simulink subsystem "Subsys_GFormConv_InnerCtrl_cascadedPI"  (R2024b)
settings: Solver=VariableStepAuto  StartTime=0.0  StopTime=10.0  RelTol=1e-3
model mask{f_n=50, L_filter_conv_pu=[ 0.0001 0.05097], C_filter_pu=[ 0.06875 0.04569 ], send_info_messages=0, K_p_V_cap_controller=0.8, K_i_V_cap_controller=0.5, K_p_I_conv_controller=3.3, K_i_I_conv_controller=16.5, Cff_V_cap_ctrl=0, Cff_I_conv_ctrl=0, K_ff_I_grid=1, K_ff_V_cap=1, i_conv_limit=1, v_conv_limit=1.3, i_lim_type=0, T_s_ctrl=1e-4, T_s_PWM_meas=1e-4, datatype='double'}
  mask prompts: f_n "Nominal frequency [Hz]"; L_filter_conv_pu "Impedance of Converter-Side Inductor [ R L ] (p.u.)"; C_filter_pu "Impedance of Filter Capacitor [ R C ] (p.u.)"; send_info_messages "Send info messages when limiting reference values (0 = disabled, 1 = enabled)"; K_p_V_cap_controller "Voltage controller proportional gain [p.u.]"; K_i_V_cap_controller "Voltage controller integral gain [p.u.]"; K_p_I_conv_controller "Current controller proportional gain [p.u.]"; K_i_I_conv_controller "Current controller integral gain [p.u.]"; Cff_V_cap_ctrl "Command-feed-forward (voltage controller) (0 = disabled, 1 = enabled)"; Cff_I_conv_ctrl "Command-feed-forward (current controller) (0 = disabled, 1 = enabled)"; K_ff_I_grid "Current-feed-forward (voltage controller) (0 = disabled, 1 = enabled)"; K_ff_V_cap "Voltage-feed-forward (current controller) (0 = disabled, 1 = enabled)"; i_conv_limit "Converter current maximum value (limit) [p.u.]"; v_conv_limit "Converter voltage maximum value (limit) [p.u.]"; i_lim_type "Coordinate system of current setpoint limiter (0 = dq, 1 = abc)"; T_s_ctrl "Controller sample time [s]"; T_s_PWM_meas "PWM and measurements sample time [s]"; datatype "Signal data type"
libraries: simulink x8
settings Model: Creator=winkens  LastModifiedBy=k.kocaogullar
settings SolverCC: AlgebraicLoopSolver=TrustRegion
settings OptimizationCC: ReuseModelBlockBuffer=off
settings DebuggingCC: UnconnectedInputMsg=warning  UnconnectedOutputMsg=warning  UnconnectedLineMsg=warning
settings ModelReferenceCC: EnableRefExpFcnMdlSchedulingChecks=on
settings RTWCC: GPUComputeCapability=3.5  DLArmComputeVersion=19.05

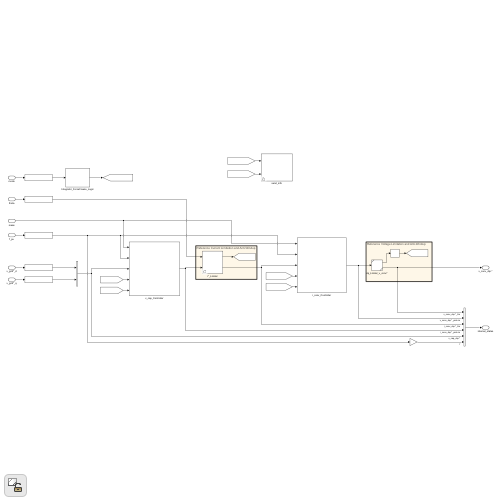
[thumbnail: Simulink's stored preview of the top-level diagram]
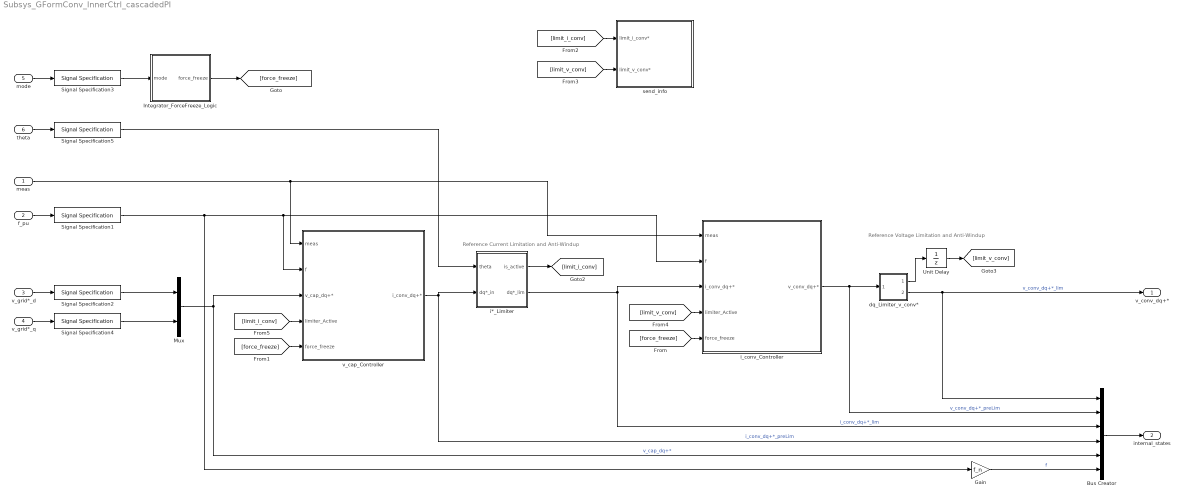
== system Subsys_GFormConv_InnerCtrl_cascadedPI ==
  note: Reference Current Limitation and Anti-Windup
  note: Reference Voltage Limitation and Anti-Windup
  meas : Inport
  f_pu : Inport  Port=2
  v_grid*_d : Inport  Port=3
  v_grid*_q : Inport  Port=4
  mode : Inport  Port=5
  theta : Inport  Port=6
  Bus Creator : BusCreator  Inputs=6
  Gain : Gain  Gain=f_n
  Integrator_ForceFreeze_Logic : Subsystem
  Mux : Mux  Inputs=2
  Signal Specification{1..4} (4 alike) : SignalSpecification  SampleTime=T_s_ctrl
  Signal Specification5 : SignalSpecification  SampleTime=T_s_PWM_meas
  Unit Delay : UnitDelay  SampleTime=-1  HasFrameUpgradeWarning=on
  dq_Limiter_v_conv* : Subsystem  ReferencedSubsystem=dq_Limiter  X_dq_max=v_conv_limit  datatype=datatype
  i*_Limiter : Subsystem  Variant=on  VariantControl=Choice
  "i_conv_Controller " : Subsystem
  send_info : Subsystem  Variant=on
  v_cap_Controller : Subsystem
  v_conv_dq+* : Outport
  internal_states : Outport  Port=2
  wires:
  Unit Delay/1 -> [limit_v_conv]
  Mux/1 -> Bus Creator/5, v_cap_Controller/3(v_cap_dq+*)  "v_cap_dq+*"
  v_grid*_d/1 -> Signal Specification2/1
  dq_Limiter_v_conv*/2 -> v_conv_dq+*/1, Bus Creator/1  "v_conv_dq+*_lim"
  f_pu/1 -> Signal Specification1/1
  v_cap_Controller/1(i_conv_dq+*) -> i*_Limiter/2(dq*_in), Bus Creator/4  "i_conv_dq+*_preLim"
  [force_freeze] -> "i_conv_Controller "/5(force_freeze)
  Gain/1 -> Bus Creator/6  "f"
  Signal Specification4/1 -> Mux/2
  dq_Limiter_v_conv*/1 -> Unit Delay/1
  "i_conv_Controller "/1(v_conv_dq+*) -> dq_Limiter_v_conv*/1, Bus Creator/2  "v_conv_dq+*_preLim"
  mode/1 -> Signal Specification3/1
  Bus Creator/1 -> internal_states/1
  meas/1 -> v_cap_Controller/1(meas), "i_conv_Controller "/1(meas)
  Signal Specification1/1 -> v_cap_Controller/2(f), "i_conv_Controller "/2(f), Gain/1
  Signal Specification2/1 -> Mux/1
  v_grid*_q/1 -> Signal Specification4/1
  theta/1 -> Signal Specification5/1
  i*_Limiter/1(is_active) -> [limit_i_conv]
  i*_Limiter/2(dq*_lim) -> Bus Creator/3, "i_conv_Controller "/3(i_conv_dq+*)  "i_conv_dq+*_lim"
  Signal Specification5/1 -> i*_Limiter/1(theta)
  [limit_i_conv] -> send_info/1(limit_i_conv*)
  [limit_v_conv] -> send_info/2(limit_v_conv*)
  Signal Specification3/1 -> Integrator_ForceFreeze_Logic/1(mode)
  Integrator_ForceFreeze_Logic/1(force_freeze) -> [force_freeze]
  [force_freeze] -> v_cap_Controller/5(force_freeze)
  [limit_v_conv] -> "i_conv_Controller "/4(limiter_Active)
  [limit_i_conv] -> v_cap_Controller/4(limiter_Active)

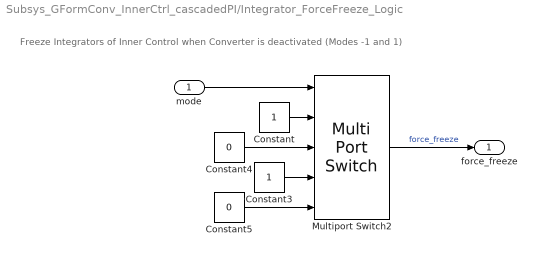
== system Subsys_GFormConv_InnerCtrl_cascadedPI/Integrator_ForceFreeze_Logic ==
  note: Freeze Integrators of Inner Control when Converter is deactivated (Modes -1 and 1)
  mode : Inport
  Constant : Constant  OutDataTypeStr=boolean
  Constant3 : Constant  OutDataTypeStr=boolean
  Constant4 : Constant  Value=0  OutDataTypeStr=boolean
  Constant5 : Constant  Value=0  OutDataTypeStr=boolean
  Multiport Switch2 : MultiPortSwitch  DataPortOrder=Specify indices  DataPortIndices={-1,0,1,2}  SaturateOnIntegerOverflow=off  InputSameDT=off
  force_freeze : Outport
  wires:
  Constant5/1 -> Multiport Switch2/5
  Constant4/1 -> Multiport Switch2/3
  Constant3/1 -> Multiport Switch2/4
  Constant/1 -> Multiport Switch2/2
  mode/1 -> Multiport Switch2/1
  Multiport Switch2/1 -> force_freeze/1  "force_freeze"

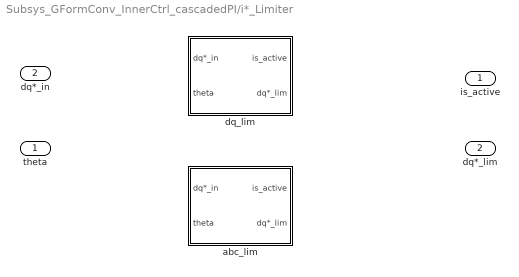
== system Subsys_GFormConv_InnerCtrl_cascadedPI/i*_Limiter ==
  theta : Inport
  dq*_in : Inport  Port=2
  abc_lim : Subsystem  VariantControl=i_lim_type > 0.5
  dq_lim : Subsystem  VariantControl=(default)
  is_active : Outport
  dq*_lim : Outport  Port=2

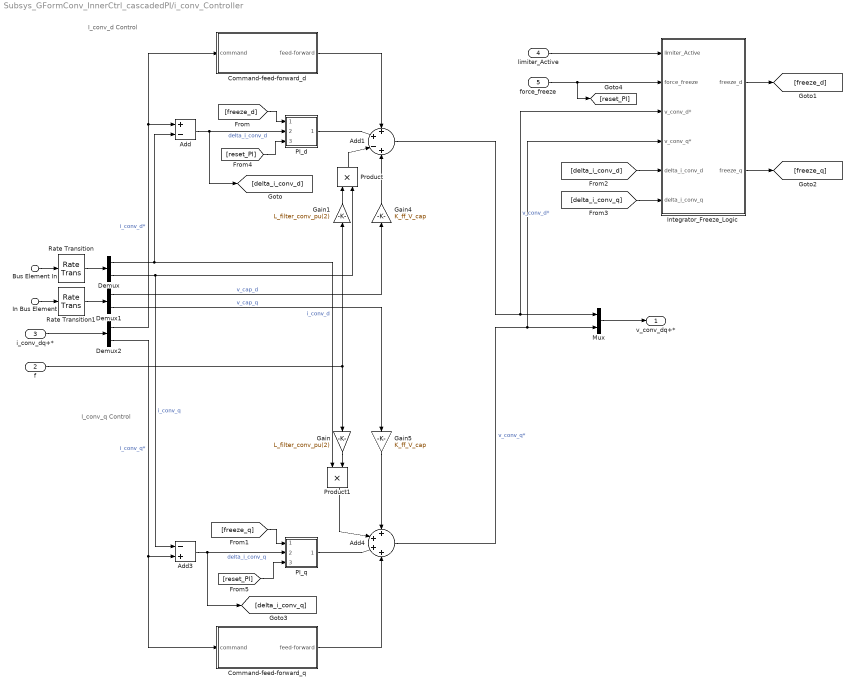
== system Subsys_GFormConv_InnerCtrl_cascadedPI/i_conv_Controller  ==
  note: I_conv_q Control
  note: I_conv_d Control
  Bus Element In : Inport  PortName=meas  Element=dq+.i_conv_dq+
  In Bus Element : Inport  PortName=meas  Element=dq+.v_cap_dq+
  f : Inport  Port=2
  i_conv_dq+* : Inport  Port=3
  limiter_Active : Inport  Port=4
  force_freeze : Inport  Port=5
  Add : Sum  Inputs=+-
  Add1 : Sum  Inputs=++-+
  Add3 : Sum  Inputs=-+
  Add4 : Sum  Inputs=++++
  Command-feed-forward_d : Subsystem  Variant=on  VariantControl=Choice
  Command-feed-forward_q : Subsystem  Variant=on  VariantControl=Choice
  Demux : Demux  Outputs=2
  Demux1 : Demux  Outputs=2
  Demux2 : Demux  Outputs=2
  Gain : Gain  Gain=L_filter_conv_pu(2)
  Gain1 : Gain  Gain=L_filter_conv_pu(2)
  Gain4 : Gain  Gain=K_ff_V_cap
  Gain5 : Gain  Gain=K_ff_V_cap
  Integrator_Freeze_Logic : Subsystem
  Mux : Mux  Inputs=2
  PI_d : Subsystem  ReferencedSubsystem=PI_freeze  K_p=K_p_I_conv_controller  K_i=K_i_I_conv_controller  T_s=T_s_ctrl  datatype=datatype
  PI_q : Subsystem  ReferencedSubsystem=PI_freeze  K_p=K_p_I_conv_controller  K_i=K_i_I_conv_controller  T_s=T_s_ctrl  datatype=datatype
  Product : Product  Inputs=**
  Product1 : Product  Inputs=**
  Rate Transition : RateTransition  Deterministic=off  OutPortSampleTime=T_s_ctrl
  Rate Transition1 : RateTransition  Deterministic=off  OutPortSampleTime=T_s_ctrl
  v_conv_dq+* : Outport
  wires:
  Add4/1 -> Integrator_Freeze_Logic/4(v_conv_q*), Mux/2  "v_conv_q*"
  Add3/1 -> PI_q/2, [delta_i_conv_q]  "delta_i_conv_q"
  Add1/1 -> Integrator_Freeze_Logic/3(v_conv_d*), Mux/1  "v_conv_d*"
  Product/1 -> Add1/3
  PI_q/1 -> Add4/3
  Mux/1 -> v_conv_dq+*/1
  Product1/1 -> Add4/2
  Gain1/1 -> Product/1
  Demux2/1 -> Add/1, Command-feed-forward_d/1(command)  "i_conv_d*"
  PI_d/1 -> Add1/2
  Demux/2 -> Add3/1, Product/2  "i_conv_q"
  f/1 -> Gain/1, Gain1/1
  Demux2/2 -> Command-feed-forward_q/1(command), Add3/2  "i_conv_q*"
  Demux1/2 -> Gain5/1  "v_cap_q"
  Bus Element In/1 -> Rate Transition/1
  i_conv_dq+*/1 -> Demux2/1
  Demux1/1 -> Gain4/1  "v_cap_d"
  Demux/1 -> Product1/1, Add/2  "i_conv_d"
  Add/1 -> PI_d/2, [delta_i_conv_d]  "delta_i_conv_d"
  In Bus Element/1 -> Rate Transition1/1
  Command-feed-forward_q/1(feed-forward) -> Add4/4
  Gain/1 -> Product1/2
  [freeze_d] -> PI_d/1
  [freeze_q] -> PI_q/1
  Gain4/1 -> Add1/4
  Gain5/1 -> Add4/1
  Command-feed-forward_d/1(feed-forward) -> Add1/1
  Rate Transition/1 -> Demux/1
  Rate Transition1/1 -> Demux1/1
  force_freeze/1 -> [reset_PI], Integrator_Freeze_Logic/2(force_freeze)
  Integrator_Freeze_Logic/1(freeze_d) -> [freeze_d]
  Integrator_Freeze_Logic/2(freeze_q) -> [freeze_q]
  limiter_Active/1 -> Integrator_Freeze_Logic/1(limiter_Active)
  [delta_i_conv_d] -> Integrator_Freeze_Logic/5(delta_i_conv_d)
  [delta_i_conv_q] -> Integrator_Freeze_Logic/6(delta_i_conv_q)
  [reset_PI] -> PI_d/3
  [reset_PI] -> PI_q/3

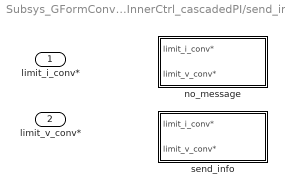
== system Subsys_GFormConv_InnerCtrl_cascadedPI/send_info ==
  limit_i_conv* : Inport
  limit_v_conv* : Inport  Port=2
  no_message : Subsystem  VariantControl=(default)
  send_info : Subsystem  VariantControl=send_info_messages > 0.5

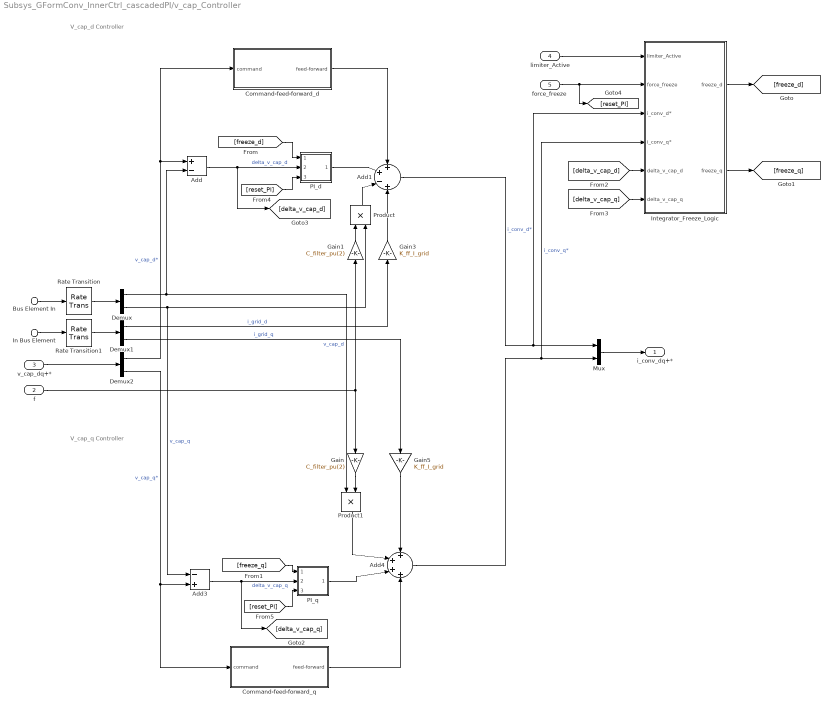
== system Subsys_GFormConv_InnerCtrl_cascadedPI/v_cap_Controller ==
  note: V_cap_q Controller
  note: V_cap_d Controller
  Bus Element In : Inport  PortName=meas  Element=dq+.v_cap_dq+
  In Bus Element : Inport  PortName=meas  Element=dq+.i_filter_grid_dq+
  f : Inport  Port=2
  v_cap_dq+* : Inport  Port=3
  limiter_Active : Inport  Port=4
  force_freeze : Inport  Port=5
  Add : Sum  Inputs=+-
  Add1 : Sum  Inputs=++-+
  Add3 : Sum  Inputs=-+
  Add4 : Sum  Inputs=++++
  Command-feed-forward_d : Subsystem  Variant=on  VariantControl=Choice
  Command-feed-forward_q : Subsystem  Variant=on  VariantControl=Choice
  Demux : Demux  Outputs=2
  Demux1 : Demux  Outputs=2
  Demux2 : Demux  Outputs=2
  Gain : Gain  Gain=C_filter_pu(2)
  Gain1 : Gain  Gain=C_filter_pu(2)
  Gain3 : Gain  Gain=K_ff_I_grid
  Gain5 : Gain  Gain=K_ff_I_grid
  Integrator_Freeze_Logic : Subsystem
  Mux : Mux  Inputs=2
  PI_d : Subsystem  ReferencedSubsystem=PI_freeze  K_p=K_p_V_cap_controller  K_i=K_i_V_cap_controller  T_s=T_s_ctrl  datatype=datatype
  PI_q : Subsystem  ReferencedSubsystem=PI_freeze  K_p=K_p_V_cap_controller  K_i=K_i_V_cap_controller  T_s=T_s_ctrl  datatype=datatype
  Product : Product  Inputs=**
  Product1 : Product  Inputs=**
  Rate Transition : RateTransition  Deterministic=off  OutPortSampleTime=T_s_ctrl
  Rate Transition1 : RateTransition  Deterministic=off  OutPortSampleTime=T_s_ctrl
  i_conv_dq+* : Outport
  wires:
  Bus Element In/1 -> Rate Transition/1
  In Bus Element/1 -> Rate Transition1/1
  v_cap_dq+*/1 -> Demux2/1
  Demux/1 -> Product1/1, Add/2  "v_cap_d"
  Demux/2 -> Add3/1, Product/2  "v_cap_q"
  Demux1/1 -> Gain3/1  "i_grid_d"
  Demux1/2 -> Gain5/1  "i_grid_q"
  Demux2/1 -> Add/1, Command-feed-forward_d/1(command)  "v_cap_d*"
  Demux2/2 -> Command-feed-forward_q/1(command), Add3/2  "v_cap_q*"
  f/1 -> Gain/1, Gain1/1
  Add/1 -> [delta_v_cap_d], PI_d/2  "delta_v_cap_d"
  PI_d/1 -> Add1/2
  Gain1/1 -> Product/1
  Product/1 -> Add1/3
  Add3/1 -> [delta_v_cap_q], PI_q/2  "delta_v_cap_q"
  PI_q/1 -> Add4/3
  Product1/1 -> Add4/2
  Gain/1 -> Product1/2
  Add1/1 -> Integrator_Freeze_Logic/3(i_conv_d*), Mux/1  "i_conv_d*"
  Add4/1 -> Integrator_Freeze_Logic/4(i_conv_q*), Mux/2  "i_conv_q*"
  Mux/1 -> i_conv_dq+*/1
  Command-feed-forward_q/1(feed-forward) -> Add4/4
  [freeze_d] -> PI_d/1
  [freeze_q] -> PI_q/1
  Gain3/1 -> Add1/4
  Gain5/1 -> Add4/1
  Command-feed-forward_d/1(feed-forward) -> Add1/1
  Rate Transition1/1 -> Demux1/1
  Rate Transition/1 -> Demux/1
  limiter_Active/1 -> Integrator_Freeze_Logic/1(limiter_Active)
  Integrator_Freeze_Logic/1(freeze_d) -> [freeze_d]
  force_freeze/1 -> [reset_PI], Integrator_Freeze_Logic/2(force_freeze)
  Integrator_Freeze_Logic/2(freeze_q) -> [freeze_q]
  [delta_v_cap_d] -> Integrator_Freeze_Logic/5(delta_v_cap_d)
  [delta_v_cap_q] -> Integrator_Freeze_Logic/6(delta_v_cap_q)
  [reset_PI] -> PI_d/3
  [reset_PI] -> PI_q/3

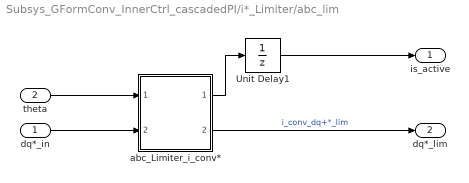
== system Subsys_GFormConv_InnerCtrl_cascadedPI/i*_Limiter/abc_lim ==
  dq*_in : Inport
  theta : Inport  Port=2
  Unit Delay1 : UnitDelay  SampleTime=-1  HasFrameUpgradeWarning=on
  abc_Limiter_i_conv* : Subsystem  ReferencedSubsystem=abc_Limiter  max_amplitude=i_conv_limit  T_s_dq=T_s_ctrl  T_s_theta=T_s_PWM_meas  datatype=datatype
  is_active : Outport
  dq*_lim : Outport  Port=2
  wires:
  abc_Limiter_i_conv*/1 -> Unit Delay1/1
  abc_Limiter_i_conv*/2 -> dq*_lim/1  "i_conv_dq+*_lim"
  Unit Delay1/1 -> is_active/1
  dq*_in/1 -> abc_Limiter_i_conv*/2
  theta/1 -> abc_Limiter_i_conv*/1

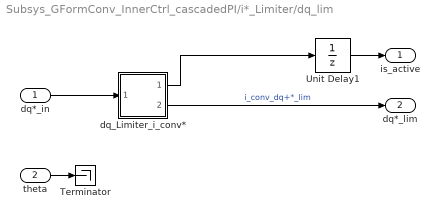
== system Subsys_GFormConv_InnerCtrl_cascadedPI/i*_Limiter/dq_lim ==
  dq*_in : Inport
  theta : Inport  Port=2
  Terminator : Terminator
  Unit Delay1 : UnitDelay  SampleTime=-1  HasFrameUpgradeWarning=on
  dq_Limiter_i_conv* : Subsystem  ReferencedSubsystem=dq_Limiter  X_dq_max=i_conv_limit  datatype=datatype
  is_active : Outport
  dq*_lim : Outport  Port=2
  wires:
  dq_Limiter_i_conv*/1 -> Unit Delay1/1
  dq_Limiter_i_conv*/2 -> dq*_lim/1  "i_conv_dq+*_lim"
  Unit Delay1/1 -> is_active/1
  dq*_in/1 -> dq_Limiter_i_conv*/1
  theta/1 -> Terminator/1

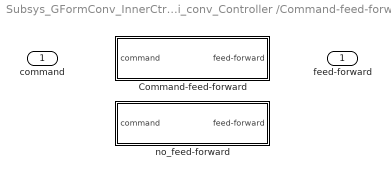
== system Subsys_GFormConv_InnerCtrl_cascadedPI/i_conv_Controller /Command-feed-forward_d ==
  command : Inport
  Command-feed-forward : Subsystem  VariantControl=Cff_I_conv_ctrl > 0.5
  no_feed-forward : Subsystem  VariantControl=(default)
  feed-forward : Outport

== system Subsys_GFormConv_InnerCtrl_cascadedPI/i_conv_Controller /Command-feed-forward_q ==
  command : Inport
  Command-feed-forward : Subsystem  VariantControl=Cff_I_conv_ctrl > 0.5
  no_feed-forward : Subsystem  VariantControl=(default)
  feed-forward : Outport

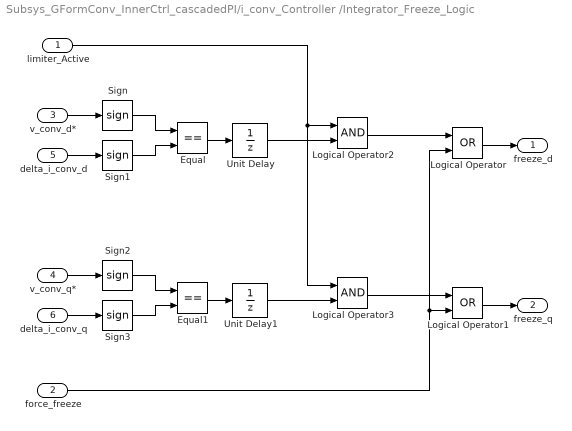
== system Subsys_GFormConv_InnerCtrl_cascadedPI/i_conv_Controller /Integrator_Freeze_Logic ==
  limiter_Active : Inport
  force_freeze : Inport  Port=2
  v_conv_d* : Inport  Port=3
  v_conv_q* : Inport  Port=4
  delta_i_conv_d : Inport  Port=5
  delta_i_conv_q : Inport  Port=6
  Equal : RelationalOperator  Operator===  OutDataTypeStr=boolean  RndMeth=Simplest  InputSameDT=off
  Equal1 : RelationalOperator  Operator===  OutDataTypeStr=boolean  RndMeth=Simplest  InputSameDT=off
  Logical Operator : Logic  Operator=OR  AllPortsSameDT=off  OutDataTypeStr=boolean
  Logical Operator1 : Logic  Operator=OR  AllPortsSameDT=off  OutDataTypeStr=boolean
  Logical Operator2 : Logic  AllPortsSameDT=off  OutDataTypeStr=boolean
  Logical Operator3 : Logic  AllPortsSameDT=off  OutDataTypeStr=boolean
  Sign{,1..3} (4 alike) : Signum
  Unit Delay : UnitDelay  SampleTime=-1  HasFrameUpgradeWarning=on
  Unit Delay1 : UnitDelay  SampleTime=-1  HasFrameUpgradeWarning=on
  freeze_d : Outport
  freeze_q : Outport  Port=2
  wires:
  Logical Operator/1 -> freeze_d/1
  Logical Operator1/1 -> freeze_q/1
  force_freeze/1 -> Logical Operator/2, Logical Operator1/2
  limiter_Active/1 -> Logical Operator3/1, Logical Operator2/1
  Logical Operator2/1 -> Logical Operator/1
  Logical Operator3/1 -> Logical Operator1/1
  v_conv_d*/1 -> Sign/1
  delta_i_conv_d/1 -> Sign1/1
  Sign/1 -> Equal/1
  Sign1/1 -> Equal/2
  Equal/1 -> Unit Delay/1
  Equal1/1 -> Unit Delay1/1
  Sign3/1 -> Equal1/2
  Sign2/1 -> Equal1/1
  delta_i_conv_q/1 -> Sign3/1
  v_conv_q*/1 -> Sign2/1
  Unit Delay/1 -> Logical Operator2/2
  Unit Delay1/1 -> Logical Operator3/2

== system Subsys_GFormConv_InnerCtrl_cascadedPI/send_info/no_message ==
  limit_i_conv* : Inport
  limit_v_conv* : Inport  Port=2
  Terminator : Terminator
  Terminator1 : Terminator
  wires:
  limit_v_conv*/1 -> Terminator1/1
  limit_i_conv*/1 -> Terminator/1

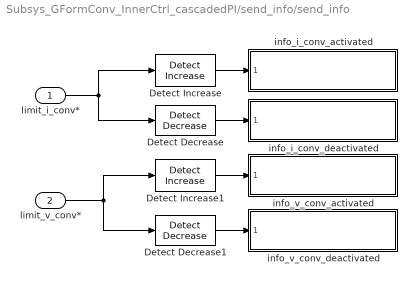
== system Subsys_GFormConv_InnerCtrl_cascadedPI/send_info/send_info ==
  limit_i_conv* : Inport
  limit_v_conv* : Inport  Port=2
  Detect Decrease : simulink/Logic and Bit Operations/Detect Decrease  vinit=0.0  OutDataTypeStr=boolean
  Detect Decrease1 : simulink/Logic and Bit Operations/Detect Decrease  vinit=0.0  OutDataTypeStr=boolean
  Detect Increase : simulink/Logic and Bit Operations/Detect Increase  vinit=0.0  OutDataTypeStr=boolean
  Detect Increase1 : simulink/Logic and Bit Operations/Detect Increase  vinit=0.0  OutDataTypeStr=boolean
  info_i_conv_activated : Subsystem  ReferencedSubsystem=tDMSquared_Info  messageText='The converter current setpoint (i_conv*) limiter is activated.'  T_s=T_s_ctrl
  info_i_conv_deactivated : Subsystem  ReferencedSubsystem=tDMSquared_Info  messageText='The converter current setpoint (i_conv*) limiter is deactivated.'  T_s=T_s_ctrl
  info_v_conv_activated : Subsystem  ReferencedSubsystem=tDMSquared_Info  messageText='The converter voltage setpoint (v_conv*) limiter is activated.'  T_s=T_s_ctrl
  info_v_conv_deactivated : Subsystem  ReferencedSubsystem=tDMSquared_Info  messageText='The converter voltage setpoint (v_conv*) limiter is deactivated.'  T_s=T_s_ctrl
  wires:
  Detect Increase/1 -> info_i_conv_activated/1
  Detect Decrease/1 -> info_i_conv_deactivated/1
  Detect Decrease1/1 -> info_v_conv_deactivated/1
  Detect Increase1/1 -> info_v_conv_activated/1
  limit_i_conv*/1 -> Detect Decrease/1, Detect Increase/1
  limit_v_conv*/1 -> Detect Decrease1/1, Detect Increase1/1

== system Subsys_GFormConv_InnerCtrl_cascadedPI/v_cap_Controller/Command-feed-forward_d ==
  command : Inport
  Command-feed-forward : Subsystem  VariantControl=Cff_V_cap_ctrl > 0.5
  no_feed-forward : Subsystem  VariantControl=(default)
  feed-forward : Outport

== system Subsys_GFormConv_InnerCtrl_cascadedPI/v_cap_Controller/Command-feed-forward_q ==
  command : Inport
  Command-feed-forward_d : Subsystem  VariantControl=Cff_V_cap_ctrl > 0.5
  no_feed-forward_d : Subsystem  VariantControl=(default)
  feed-forward : Outport

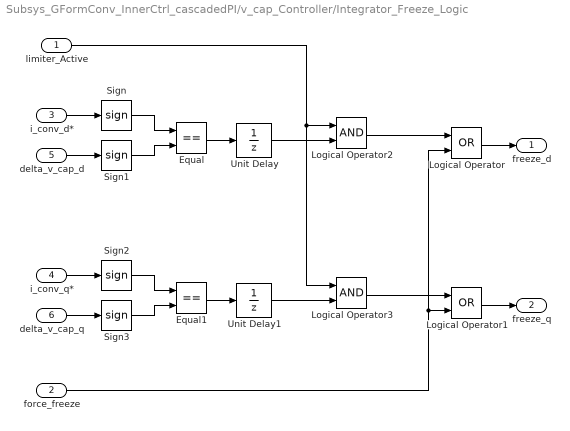
== system Subsys_GFormConv_InnerCtrl_cascadedPI/v_cap_Controller/Integrator_Freeze_Logic ==
  limiter_Active : Inport
  force_freeze : Inport  Port=2
  i_conv_d* : Inport  Port=3
  i_conv_q* : Inport  Port=4
  delta_v_cap_d : Inport  Port=5
  delta_v_cap_q : Inport  Port=6
  Equal : RelationalOperator  Operator===  OutDataTypeStr=boolean  RndMeth=Simplest  InputSameDT=off
  Equal1 : RelationalOperator  Operator===  OutDataTypeStr=boolean  RndMeth=Simplest  InputSameDT=off
  Logical Operator : Logic  Operator=OR  AllPortsSameDT=off  OutDataTypeStr=boolean
  Logical Operator1 : Logic  Operator=OR  AllPortsSameDT=off  OutDataTypeStr=boolean
  Logical Operator2 : Logic  AllPortsSameDT=off  OutDataTypeStr=boolean
  Logical Operator3 : Logic  AllPortsSameDT=off  OutDataTypeStr=boolean
  Sign{,1..3} (4 alike) : Signum
  Unit Delay : UnitDelay  SampleTime=-1  HasFrameUpgradeWarning=on
  Unit Delay1 : UnitDelay  SampleTime=-1  HasFrameUpgradeWarning=on
  freeze_d : Outport
  freeze_q : Outport  Port=2
  wires:
  Logical Operator/1 -> freeze_d/1
  Logical Operator1/1 -> freeze_q/1
  force_freeze/1 -> Logical Operator/2, Logical Operator1/2
  limiter_Active/1 -> Logical Operator3/1, Logical Operator2/1
  Logical Operator2/1 -> Logical Operator/1
  Logical Operator3/1 -> Logical Operator1/1
  i_conv_d*/1 -> Sign/1
  delta_v_cap_d/1 -> Sign1/1
  Sign/1 -> Equal/1
  Sign1/1 -> Equal/2
  Equal/1 -> Unit Delay/1
  Equal1/1 -> Unit Delay1/1
  Sign3/1 -> Equal1/2
  Sign2/1 -> Equal1/1
  delta_v_cap_q/1 -> Sign3/1
  i_conv_q*/1 -> Sign2/1
  Unit Delay/1 -> Logical Operator2/2
  Unit Delay1/1 -> Logical Operator3/2

== system Subsys_GFormConv_InnerCtrl_cascadedPI/i_conv_Controller /Command-feed-forward_d/Command-feed-forward ==
  command : Inport
  Discrete Derivative1 : simulink/Discrete/Discrete Derivative  gainval=1.0  ICPrevScaledInput=0.0  OutMin=[]  OutMax=[]  OutDataType=fixdt(1, 16)  OutScaling=2^-10  DoSatur=off
  Gain2 : Gain  Gain=L_filter_conv_pu(2)
  feed-forward : Outport
  wires:
  Discrete Derivative1/1 -> Gain2/1
  command/1 -> Discrete Derivative1/1
  Gain2/1 -> feed-forward/1

== system Subsys_GFormConv_InnerCtrl_cascadedPI/i_conv_Controller /Command-feed-forward_d/no_feed-forward ==
  command : Inport
  Ground : Ground
  Terminator : Terminator
  feed-forward : Outport
  wires:
  Ground/1 -> feed-forward/1
  command/1 -> Terminator/1

== system Subsys_GFormConv_InnerCtrl_cascadedPI/i_conv_Controller /Command-feed-forward_q/Command-feed-forward ==
  command : Inport
  Discrete Derivative1 : simulink/Discrete/Discrete Derivative  gainval=1.0  ICPrevScaledInput=0.0  OutMin=[]  OutMax=[]  OutDataType=fixdt(1, 16)  OutScaling=2^-10  DoSatur=off
  Gain2 : Gain  Gain=L_filter_conv_pu(2)
  feed-forward : Outport
  wires:
  Discrete Derivative1/1 -> Gain2/1
  command/1 -> Discrete Derivative1/1
  Gain2/1 -> feed-forward/1

== system Subsys_GFormConv_InnerCtrl_cascadedPI/i_conv_Controller /Command-feed-forward_q/no_feed-forward ==
  command : Inport
  Ground : Ground
  Terminator : Terminator
  feed-forward : Outport
  wires:
  Ground/1 -> feed-forward/1
  command/1 -> Terminator/1

== system Subsys_GFormConv_InnerCtrl_cascadedPI/v_cap_Controller/Command-feed-forward_d/Command-feed-forward ==
  command : Inport
  Discrete Derivative1 : simulink/Discrete/Discrete Derivative  gainval=1.0  ICPrevScaledInput=0.0  OutMin=[]  OutMax=[]  OutDataType=fixdt(1, 16)  OutScaling=2^-10  DoSatur=off
  Gain2 : Gain  Gain=C_filter_pu(2)
  feed-forward : Outport
  wires:
  Discrete Derivative1/1 -> Gain2/1
  command/1 -> Discrete Derivative1/1
  Gain2/1 -> feed-forward/1

== system Subsys_GFormConv_InnerCtrl_cascadedPI/v_cap_Controller/Command-feed-forward_d/no_feed-forward ==
  command : Inport
  Ground : Ground
  Terminator : Terminator
  feed-forward : Outport
  wires:
  Ground/1 -> feed-forward/1
  command/1 -> Terminator/1

== system Subsys_GFormConv_InnerCtrl_cascadedPI/v_cap_Controller/Command-feed-forward_q/Command-feed-forward_d ==
  command : Inport
  Discrete Derivative1 : simulink/Discrete/Discrete Derivative  gainval=1.0  ICPrevScaledInput=0.0  OutMin=[]  OutMax=[]  OutDataType=fixdt(1, 16)  OutScaling=2^-10  DoSatur=off
  Gain2 : Gain  Gain=C_filter_pu(2)
  feed-forward : Outport
  wires:
  Discrete Derivative1/1 -> Gain2/1
  command/1 -> Discrete Derivative1/1
  Gain2/1 -> feed-forward/1

== system Subsys_GFormConv_InnerCtrl_cascadedPI/v_cap_Controller/Command-feed-forward_q/no_feed-forward_d ==
  command : Inport
  Ground : Ground
  Terminator : Terminator
  feed-forward : Outport
  wires:
  Ground/1 -> feed-forward/1
  command/1 -> Terminator/1
